simulink model "QD2_DroneStack_MPC"  (R2022b)
settings: Solver=ode1  StartTime=0.0  StopTime=inf  FixedStep=1/1000  RelTol=1e-3  EnableMultiTasking=on
InitFcn:
  | % QD2_DroneStack_MPC: rutas de la librería qd2_* y del mapeo de motores
  | qd2_d = fileparts(get_param(bdroot, 'FileName'));
  | for qd2_k = 1:4
  |     if exist(fullfile(qd2_d, 'lib', 'qd2_params.m'), 'file'), break; end
  |     qd2_d = fileparts(qd2_d);
  | end
  | addpath(fullfile(qd2_d, 'lib'));
  | addpath(fullfile(qd2_d, 'equipo2_original'));
  | clear qd2_d qd2_k
  | Motor_Mapping_7_Inch
model workspace (MAT data in the model file):
  target_system = 1
undefined symbols (not defined in the file): _Commander, _QDrone2, _Stabilizer, datetime, HIL, KT, lf, log_, m, Motor_Matrix, n, qc_get_step_size, s, saved_data
libraries: quarc_library x94, simulink x27, simulink_extras x9
(part 2 of 5)

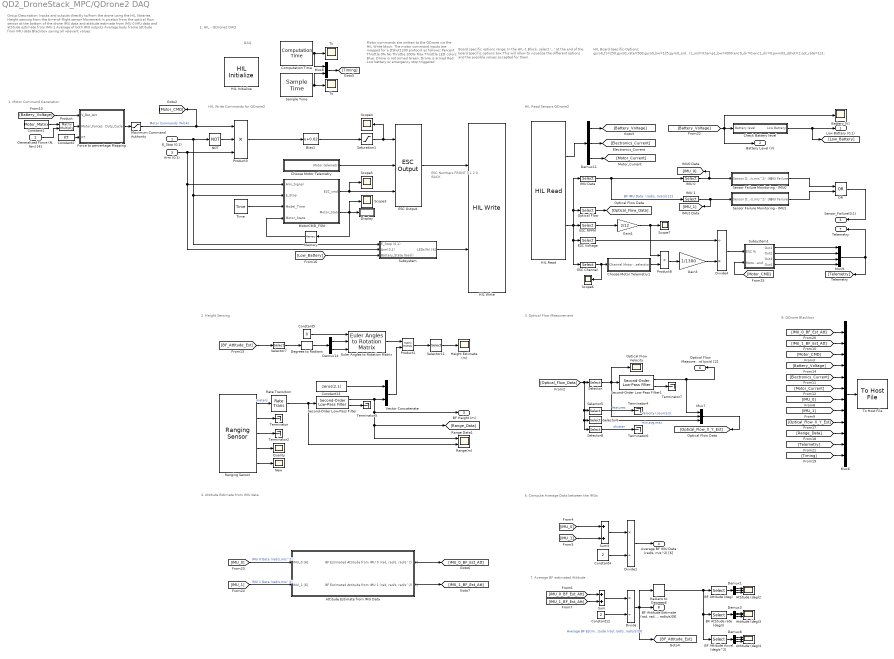
== system QD2_DroneStack_MPC/QDrone2 DAQ ==
  note: 4. Attitude Estimate from IMU data
  note: 1. Motor Command Generation
  note: HIL Write Commands for QDrone2
  note: HIL Read Sensors QDrone2
  note: ESC Numbers
      |
      | FRONT
      | 3 1
      |
      | 2 0
      | BACK
  note: 1. HIL - QDrone2 DAQ
  note: Group Description:
      |
      | Inputs and outputs directly to/from the drone using the HIL libraries.
      | Height sensing from the time-of-flight sensor
      | Movement in pixels/s from the optical flow sensor at the bottom of the drone
      | IMU data and attitude estimate from IMU 0
      | IMU data and attitude estimate from IMU 1
      | Average of both IMU outputs
      | Average body frame attitude from IMU data
      | Blackbox saving all relevant values
  note: DAQ
  note: HIL Board Specific-Options:
      | gyro0_fs=250;gyro0_rate=500;gyro0_bw=125;gyro0_ord=3;accel0_fs=16;accel0_rate=1000;accel0_bw=400;accel0_ord=3;temp0_bw=4000;gyro1_fs=250;gyro1_rate=500;gyro1_bw=125;gyro1_ord=3;accel1_fs=16;accel1_rate=1000;accel1_bw=400;accel1_ord=3;temp1_bw=4000;enc0_dir=0;enc1_dir=0;pwm03_dshot=1;opt_rate=121;
  note: Motor commands are written to the QDrone via the HIL Write block. The motor command inputs are mapped for a DShot1200 protocol as follows:
      |
      | Percent Throttle
      | 0% No Throttle
      | 100% Max Throttle
      |
      | LED colors:
      | Blue: Drone is not armed
      | Green: Drone is armed
      | Red: Low battery or emergency stop triggered
  note: Board specific options range:
      |
      | In the HIL-1 Block,
      | select '...' at the end of the board specific options box
      | This will allow to visualize the different options
      | and the possible values accepted for them.
  note: 2. Height Sensing
  note: 8. QDrone Blackbox
  note: 6. Compute Average Data between the IMUs
  note: 7. Average BF estimated Attitude
  note: 3. Optical Flow Measurement
  E_Stop (0,1) : Inport
  "Generalized Force (N, Nm) [4]" : Inport  Port=2
  Arm (0,1) : Inport  Port=3
  Attitude (deg)2 : Scope  NumInputPorts=3
  Attitude (deg)3 : Scope  NumInputPorts=3
  Attitude (deg)4 : Scope  NumInputPorts=3
  Attitude Estimate from IMU Data : Subsystem
  BF Attitude (deg) : Selector  InputPortWidth=9  IndexOptions=Index vector (dialog)  Indices=[1:3]  OutputSizes=1
  BF Attitude Accel (deg/s^2) : Selector  InputPortWidth=9  IndexOptions=Index vector (dialog)  Indices=[7:9]  OutputSizes=1
  BF Attitude rate (deg/s) : Selector  InputPortWidth=9  IndexOptions=Index vector (dialog)  Indices=[4:6]  OutputSizes=1
  Battery (V) : Scope
  Bias1 : Bias  Bias=0.02  SaturateOnIntegerOverflow=off
  Check Battery level : Subsystem
  Choose Motor Telemetry : Subsystem
  Choose Motor Telemetry1 : Subsystem
  Computation Time : quarc_library/Sources/Time/Computation Time  sample_time=qc_get_step_size  use_model=on  use_cpu_time=off
  Constant1 : Constant  Value=Motor_Matrix  OutDataTypeStr=double
  Constant12 : Constant  Value=2
  Constant13 : Constant  Value=zeros(2,1)
  Constant2 : Constant  Value=KT  OutDataTypeStr=double
  Constant4 : Constant  Value=2
  Constant5 : Constant  Value=0
  Degrees to Radians : simulink_extras/Transformations/Degrees to Radians
  Demux{1,3,8,11} (4 alike) : Demux  Outputs=3
  Demux14 : Demux  Outputs=2
  Display : Display
  Divide : Product  Inputs=*/
  Divide1 : Product  Inputs=*/
  Divide4 : Product  Inputs=/*
  ESC Channel : Selector  InputPortWidth=22  IndexOptions=Index vector (dialog)  Indices=[22]  OutputSizes=1
  ESC Output : quarc_library/Data Acquisition/Generic/Transformations/ESC Output  protocol=DShot (raw)  sign=Unsigned
      settings: AttributesFormatString=%<protocol>  SourceProductName=QUARC Targets
  ESC RPPM : Selector  InputPortWidth=22  IndexOptions=Index vector (dialog)  Indices=[20]  OutputSizes=1
  ESC Voltage : Selector  InputPortWidth=22  IndexOptions=Index vector (dialog)  Indices=[21]  OutputSizes=1
  Euler Angles to Rotation Matrix : quarc_library/Math Operations/Matrices/Euler Angles to Rotation Matrix  menu_order=Relative Z-X-Y
      settings: SourceProductName=QUARC Targets
  Force to percentage Mapping : MATLAB Function  TreatAsAtomicUnit=on
  Gain1 : Gain  Gain=2/12
  Gain3 : Gain  Gain=1/1300
  HIL Initialize : quarc_library/Data Acquisition/Generic/Configuration/HIL Initialize  object_name=HIL-1  board_type=qdrone2  board_number=0  board_options=gyro0_fs=250;gyro0_rate=500;gyro0_bw=125;gyro0_ord=3;accel0_fs=16;accel0_rate=1000;accel0_bw=400;accel0_ord=3;temp0_bw=4000;gyro1_fs=250;gyro1_rate=500;gyro1_bw=125;gyro1_ord=3;accel1_fs=16;accel1_rate=1000;accel1_bw=400;accel1_ord=3;temp1_bw=4000;enc0_dir=0;enc1_dir=0;pwm03_dshot=1;opt_rate=121;  exclusive=off  active=on  hardware_clocks=[]  clock_modes=[]  initial_clock_frequencies=[]  set_clock_params_at_start=off  set_clock_params_at_switch_in=off  set_clock_frequencies_at_start=off  set_clock_frequencies_at_switch_in=off  analog_input_channels=[0:4]  analog_input_configurations=[]  analog_input_maximums=[3.3]  analog_input_minimums=[0]  set_analog_input_params_at_start=off  set_analog_input_params_at_switch_in=off  analog_output_channels=[]  analog_output_maximums=[]  analog_output_minimums=[]  initial_analog_outputs=[]  final_analog_outputs=[]  watchdog_analog_outputs=[]  set_analog_output_params_at_start=off  set_analog_output_params_at_switch_in=off  set_analog_outputs_at_start=off  set_analog_outputs_at_switch_in=off  set_analog_outputs_at_terminate=off  set_analog_outputs_at_switch_out=off  set_analog_outputs_on_watchdog=off  digital_input_channels=[0:5]  digital_output_channels=[6:11]  digital_output_configuration=[]  initial_digital_outputs=[0]  final_digital_outputs=[0]  watchdog_digital_outputs=[0 0 0 0 0 0]  set_digital_output_params_at_start=off  set_digital_output_params_at_switch_in=off  set_digital_outputs_at_start=on  set_digital_outputs_at_switch_in=off  set_digital_outputs_at_terminate=on  set_digital_outputs_at_switch_out=off  set_digital_outputs_on_watchdog=off  encoder_channels=[0:1]  quadrature=[4]  encoder_filter_frequency=100e6/1  initial_encoder_counts=[0]  set_encoder_params_at_start=on  set_encoder_params_at_switch_in=off  set_encoder_counts_at_start=on  set_encoder_counts_at_switch_in=off  pwm_channels=[0:5]  pwm_modes=[6 6 6 6 0 0]  pwm_frequency=1.2e6  pwm_configuration=[0]  pwm_alignment=[0]  pwm_polarity=[1]  pwm_leading_deadband=[]  pwm_trailing_deadband=[]  initial_pwm_outputs=[0]  final_pwm_outputs=[0]  watchdog_pwm_outputs=[0]  set_pwm_params_at_start=on  set_pwm_params_at_switch_in=off  set_pwm_outputs_at_start=on  set_pwm_outputs_at_switch_in=off  set_pwm_outputs_at_terminate=on  set_pwm_outputs_at_switch_out=off  set_pwm_outputs_on_watchdog=off  other_output_channels=[]  initial_other_outputs=[0]  final_other_outputs=[0]  watchdog_other_outputs=[]  set_other_outputs_at_start=on  set_other_outputs_at_switch_in=off  set_other_outputs_at_terminate=on  set_other_outputs_at_switch_out=off  set_other_outputs_on_watchdog=off
  HIL Read : quarc_library/Data Acquisition/Generic/Immediate I//O/HIL Read  object_name=HIL-1  analog_channels=[3 1:2]  encoder_channels=[]  digital_channels=[]  other_channels=[3000:3002 4000:4002 3003:3005 4003:4005 17000:17006 17008:17009 17007]  sample_time=qc_get_step_size  active=on  vector_output=on  port_labels=channel numbers  data_type_mode=Inherit via back propagation  encoder_data_type=double  digital_data_type=boolean
  HIL Write : quarc_library/Data Acquisition/Generic/Immediate I//O/HIL Write  object_name=HIL-1  analog_channels=[]  pwm_channels=[0:3]  digital_channels=[6:11]  other_channels=[]  sample_time=-1  active=off  vector_input=on  port_labels=channel numbers
  Height Estimate (m) : Scope
  IMU 0 : Selector  InputPortWidth=12  IndexOptions=Index vector (dialog)  Indices=[1:6]  OutputSizes=1
  IMU 1 : Selector  InputPortWidth=12  IndexOptions=Index vector (dialog)  Indices=[7:12]  OutputSizes=1
  IMU Data : Selector  InputPortWidth=22  IndexOptions=Index vector (dialog)  Indices=[1:12]  OutputSizes=1
  "Maximum Command Authority " : Saturate  UpperLimit=[1 1 1 1]  LowerLimit=[0 0 0 0]
  Memory : Memory
  MotorCMD_FSM : MATLAB Function  TreatAsAtomicUnit=on
  Mux6 : Mux  Inputs=12
  Mux7 : Mux  Inputs=3
  Mux8 : Mux  Inputs=2
  Mux9 : Mux
  NOT : Logic  Operator=NOT  IconShape=distinctive  AllPortsSameDT=off  OutDataTypeStr=boolean
  New : Scope
  OR : Logic  Operator=OR  AllPortsSameDT=off  OutDataTypeStr=boolean
  Optical Flow : Selector  InputPortWidth=22  IndexOptions=Index vector (dialog)  Indices=[13:19]  OutputSizes=1
  Optical Flow Velocity : Scope
  Product : Product  Multiplication=Matrix(*)
  Product1 : Product  Multiplication=Matrix(*)
  Product3 : Product  Inputs=3
  Product8 : Product
  Quality : Scope
  Radians to Degrees6 : simulink_extras/Transformations/Radians to Degrees
  Range(m) : Scope  NumInputPorts=2
  Ranging Sensor : quarc_library/Devices/Third-Party/Sensors/Ranging Sensor  sensor_type=VL53L1X Time-of-flight  uri=i2c-cpu://localhost:0?address='0x29',baud='400000',memsize='512'  ranging_distance=Long  timing_budget=0.033  measurement_period=0.040  output_mode=Fixed-size output  samples_per_revolution=1300  max_distance=0.050  max_angle=5  sample_time=qc_get_step_size * ceil(1/121/ qc_get_step_size)  show_versions=off  active=on
      settings: SourceProductName=QUARC Targets
  Rate Transition : RateTransition
  Sample Time : quarc_library/Sources/Time/Sample Time  Priority=-99  sample_time=qc_get_step_size
  Saturation1 : Saturate  UpperLimit=1  LowerLimit=0
  Scope{3..7} (5 alike) : Scope
  Second-Order Low-Pass Filter : quarc_library/Continuous/Second-Order Low-Pass Filter  params_source=Internal (dialog parameters)  input_width=100  input_zeta=0.7  input_init=0
  Second-Order Low-Pass Filter1 : quarc_library/Continuous/Second-Order Low-Pass Filter  params_source=Internal (dialog parameters)  input_width=45  input_zeta=1.5  input_init=0
  Selector : Selector  InputPortWidth=7  IndexOptions=Index vector (dialog)  Indices=[1 2]  OutputSizes=1
  Selector11 : Selector  InputPortWidth=3  IndexOptions=Index vector (dialog)  Indices=[3]  OutputSizes=1
  Selector5 : Selector  InputPortWidth=7  IndexOptions=Index vector (dialog)  Indices=[3]  OutputSizes=1
  Selector6 : Selector  InputPortWidth=7  IndexOptions=Index vector (dialog)  Indices=[4 5 6]  OutputSizes=1
  Selector7 : Selector  InputPortWidth=9  IndexOptions=Index vector (dialog)  Indices=[1,2]  OutputSizes=1
  Selector8 : Selector  InputPortWidth=7  IndexOptions=Index vector (dialog)  Indices=[7]  OutputSizes=1
  Sensor Failure Monitoring - IMU0 : Subsystem
  Sensor Failure Monitoring - IMU1 : Subsystem
  Subsystem : Subsystem
  Subsystem1 : Subsystem
  Sum : Sum
  Sum3 : Sum
  Tc : Scope
  Terminator{,2,4..7} (6 alike) : Terminator
  Time : quarc_library/Sources/Time/Time  time_source=Wall clock  sample_time=qc_get_step_size
  To Host File : quarc_library/Sinks/To Host/To Host File  source=Specify via dialog (do not evaluate)  file_name=saved_data/%m/log_%{regexprep(char(datetime),' ','_')}_QDrone2.mat  variable_name=QDrone_data  decimation=1  sample_time=-1  file_format=MAT-file v.4  options=No header or footer  append=off  final_file_name=saved_data/QD2_DroneStack_MPC/log_22-Nov-2026_07-15-10_QDrone2.mat  encoding=Default  bitrate=2000000
  Ts : Scope
  Vector Concatenate : Concatenate
  Low Battery (0,1) : Outport
  Battery Level (V) : Outport  Port=2
  Sensor_Failure(0,1) : Outport  Port=3
  "Average BF IMU Data (rad/s, m/s^2) [6]" : Outport  Port=4
  "BF Height (m) " : Outport  Port=5
  Optical Flow Measurement (px/s) [2] : Outport  Port=6
  Telemetry : Outport  Port=7
  "BF Attitude Estimate (rad, rad/s, rad/s/s)[9]" : Outport  Port=8
  wires:
  Constant2/1 -> Force to percentage Mapping/3(KT)
  Constant1/1 -> Product/1
  "Generalized Force (N, Nm) [4]"/1 -> Product/2
  Product/1 -> Force to percentage Mapping/2(Motor_Forces)
  Force to percentage Mapping/1(Duty_Cycle) -> "Maximum Command Authority "/1
  "Maximum Command Authority "/1 -> Product3/1, [Motor_CMD]  "Motor Commands (%)[4]"
  [Battery_Voltage] -> Force to percentage Mapping/1(V_Bat_Act)
  Bias1/1 -> Saturation1/1
  ESC Voltage/1 -> Divide4/1
  IMU 0/1 -> Sensor Failure Monitoring - IMU0/1(Sensor Data (rad/s,m/s^2)  [6]), [IMU_0]
  OR/1 -> Sensor_Failure(0,1)/1
  Check Battery level/1(Low Battery) -> [Low_Battery], Low Battery (0,1)/1
  Optical Flow/1 -> [Optical_Flow_Data]
  IMU Data/1 -> IMU 0/1, IMU 1/1  "BF IMU Data  (rad/s, m/s/s)[12]"
  HIL Read/1 -> Demux11/1
  Gain1/1 -> Product8/1, Scope7/1
  NOT/1 -> Product3/2
  Memory/1 -> MotorCMD_FSM/4("Motor_State ")
  E_Stop (0,1)/1 -> Subsystem/1(E_Stop (0,1)), MotorCMD_FSM/2(E_Stop), NOT/1
  Subsystem/1(LEDs(%) [6]) -> HIL Write/2
  Demux11/2 -> [Electronics_Current]
  Sensor Failure Monitoring - IMU0/1(IMU Failure) -> OR/1
  ESC Output/1 -> HIL Write/1
  HIL Read/2 -> IMU Data/1, Optical Flow/1, ESC Voltage/1, ESC Channel/1, ESC RPPM/1
  [Battery_Voltage] -> Check Battery level/1(Battery level), Battery Level (V)/1, Battery (V)/1
  Demux11/3 -> [Motor_Current]
  IMU 1/1 -> [IMU_1], Sensor Failure Monitoring - IMU1/1(Sensor Data (rad/s,m/s^2)  [6])
  Choose Motor Telemetry1/1(Motor selection) -> Product8/2
  MotorCMD_FSM/2(Motor_State) -> Scope3/1, Display/1, Memory/1
  Gain3/1 -> Divide4/2
  Time/1 -> MotorCMD_FSM/3(Model_Time)
  Choose Motor Telemetry/1(Motor telemetry) -> ESC Output/2
  ESC Channel/1 -> Scope6/1, Choose Motor Telemetry1/1(Channel)
  Arm (0,1)/1 -> MotorCMD_FSM/1(Arm_Signal), Subsystem/2("Arm(0,1) "), Product3/3
  MotorCMD_FSM/1(ESC_cmd) -> Scope5/1, ESC Output/3
  Sensor Failure Monitoring - IMU1/1(IMU Failure) -> OR/2
  [Low_Battery] -> Subsystem/3(Battery_State (bool))
  ESC RPPM/1 -> Gain1/1
  Product8/1 -> Gain3/1
  Product3/1 -> Bias1/1
  Saturation1/1 -> ESC Output/1, Scope4/1
  Mux8/1 -> [Timing]
  Computation Time/1 -> Mux8/1, Tc/1
  Sample Time/1 -> Mux8/2, Ts/1
  Ranging Sensor/5 -> New/1
  [Range_Data] -> Mux6/10
  Selector5/1 -> Terminator4/1  "features"
  Mux7/1 -> [Optical_Flow_X_Y_Est]
  [Motor_CMD] -> Mux6/3
  Constant12/1 -> Divide/2
  Demux14/1 -> Euler Angles to Rotation Matrix/2
  Demux3/3 -> Attitude (deg)3/3
  Demux14/2 -> Euler Angles to Rotation Matrix/3
  [IMU_0_BF_Est_Att] -> Mux6/1
  [IMU_1_BF_Est_Att] -> Sum/2
  Mux9/1 -> [Telemetry], Telemetry/1
  [Optical_Flow_Data] -> Selector8/1, Selector6/1, Selector5/1, Selector/1
  BF Attitude Accel (deg/s^2)/1 -> Demux8/1
  Divide1/1 -> "Average BF IMU Data (rad/s, m/s^2) [6]"/1
  Subsystem1/4(Out4) -> Mux9/4
  [Timing] -> Mux6/12
  Selector6/1 -> Mux7/3  "min,avg,max"
  [Motor_CMD] -> Subsystem1/2(Motor command)
  [Telemetry] -> Mux6/11
  [IMU_1_BF_Est_Att] -> Mux6/2
  Constant13/1 -> Vector Concatenate/1
  [IMU_0] -> Sum3/1
  BF Attitude rate (deg/s)/1 -> Demux3/1
  Product1/1 -> Selector11/1
  [Motor_Current] -> Mux6/6
  Selector11/1 -> Height Estimate (m)/1
  Second-Order Low-Pass Filter/1 -> Vector Concatenate/2, [Range_Data], Range(m)/1, "BF Height (m) "/1
  Demux1/2 -> Attitude (deg)2/2
  Selector7/1 -> Degrees to Radians/1
  Constant5/1 -> Euler Angles to Rotation Matrix/1
  Second-Order Low-Pass Filter1/1 -> Mux7/1, Optical Flow Measurement (px/s) [2]/1
  Rate Transition/1 -> Range(m)/2, Second-Order Low-Pass Filter/1
  Subsystem1/3(Out3) -> Mux9/3
  Demux8/3 -> Attitude (deg)4/3
  Ranging Sensor/1 -> Rate Transition/1  "meters"
  Divide/1 -> "BF Attitude Estimate (rad, rad/s, rad/s/s)[9]"/1, [BF_Attitude_Est], Radians to Degrees6/1  "Average BF Estimated Attitude (rad, rad/s, rad/s/s)[9]"
  Degrees to Radians/1 -> Demux14/1
  Constant4/1 -> Divide1/2
  Euler Angles to Rotation Matrix/1 -> Product1/1
  [IMU_1] -> Sum3/2
  Demux1/3 -> Attitude (deg)2/3
  Demux8/2 -> Attitude (deg)4/2
  [IMU_1] -> Mux6/8
  [Optical_Flow_X_Y_Est] -> Mux6/9
  [BF_Attitude_Est] -> Selector7/1
  Ranging Sensor/4 -> Quality/1
  Subsystem1/1(Out1) -> Mux9/1
  Sum/1 -> Divide/1
  Vector Concatenate/1 -> Product1/2
  Demux3/1 -> Attitude (deg)3/1
  Selector8/1 -> Terminator6/1  "shutter"
  Radians to Degrees6/1 -> BF Attitude Accel (deg/s^2)/1, BF Attitude rate (deg/s)/1, BF Attitude (deg)/1
  Demux8/1 -> Attitude (deg)4/1
  Demux3/2 -> Attitude (deg)3/2
  Ranging Sensor/2 -> Terminator/1
  Ranging Sensor/3 -> Terminator2/1
  [IMU_0] -> Mux6/7
  Demux1/1 -> Attitude (deg)2/1
  [Battery_Voltage] -> Mux6/4
  Mux6/1 -> To Host File/1
  [Electronics_Current] -> Mux6/5
  [IMU_0_BF_Est_Att] -> Sum/1
  Divide4/1 -> Subsystem1/1(ESC %)
  BF Attitude (deg)/1 -> Demux1/1
  Sum3/1 -> Divide1/1
  Subsystem1/2(Out2) -> Mux9/2
  Selector/1 -> Second-Order Low-Pass Filter1/1, Mux7/2, Optical Flow Velocity/1  "Velocity (counts/s)"
  Demux11/1 -> [Battery_Voltage]
  Second-Order Low-Pass Filter/2 -> Terminator5/1
  Second-Order Low-Pass Filter1/2 -> Terminator7/1
  [IMU_0] -> Attitude Estimate from IMU Data/1(IMU_0 [6])  "IMU 0 Data (rad/s,m/s^2)"
  [IMU_1] -> Attitude Estimate from IMU Data/2(IMU_1 [6])  "IMU 1 Data (rad/s,m/s^2)"
  Attitude Estimate from IMU Data/1("BF Estimated Attitude from IMU 0 (rad, rad/s, rad/s^2) [9]") -> [IMU_0_BF_Est_Att]
  Attitude Estimate from IMU Data/2("BF Estimated Attitude from IMU 1 (rad, rad/s, rad/s^2) [9]") -> [IMU_1_BF_Est_Att]

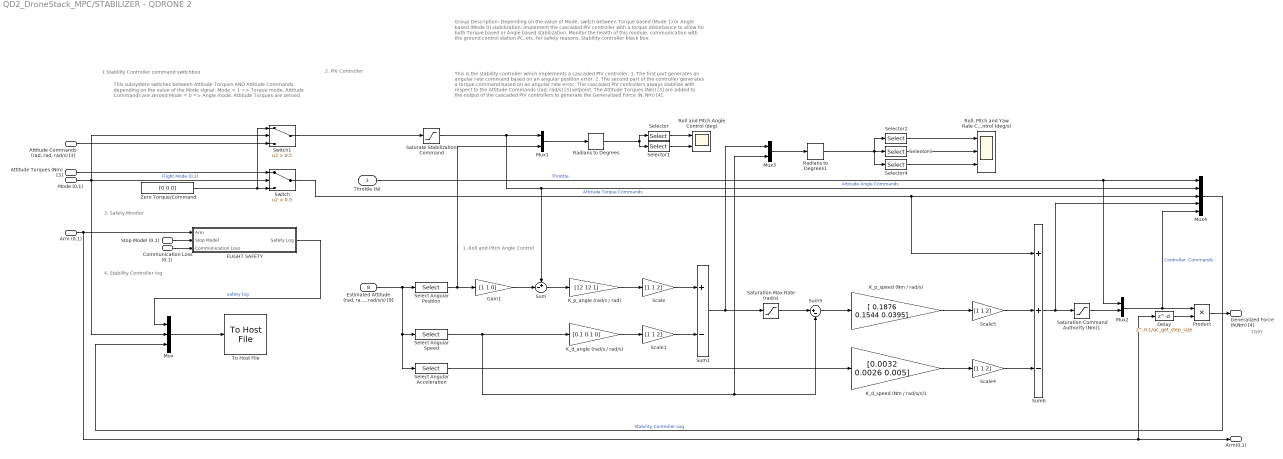
== system QD2_DroneStack_MPC/STABILIZER - QDRONE 2 ==
  note: 3. Safety Monitor
  note: This subsystem switches between Attitude Torques AND Attitude Commands depending on
      | the value of the Mode signal:
      | Mode = 1	=> 		Torque mode, Attitude Commands are zeroed
      | Mode = 0	=> 		Angle mode, Attitude Torques are zeroed
  note: This is the stability controller which implements a cascaded PIV controller.
      | 1. The first part generates an angular rate command based on an angular position error.
      | 2. The second part of the controller generates a torque command based on an angular rate error.
      |
      | The cascaded PIV controllers always stabilize with respect to the Attitude Commands (rad, rad/s) [3] setpoint. The Attitude Torques (Nm) [3] are added to the output of the cascaded PIV controllers to generate the Generalized Force (N, Nm) [4].
  note: 1. Roll and Pitch Angle Control
  note: TRPY
  note: Group Description:
      |
      | Depending on the value of Mode, switch between Torque based (Mode 1) or Angle based (Mode 0) stabilization.
      | Implement the cascaded PIV controller with a torque disturbance to allow for both Torque based or Angle based stabilization.
      | Monitor the health of this module, communication with the ground control station PC, etc. for safety reasons.
      | Stability controller black box.
  note: 1 Stability Controller command switchbox
  note: 4. Stability Controller log
  note: 2. PIV Controller
  Mode (0,1) : Inport
  Stop Model (0,1) : Inport  Port=2
  Throttle (N) : Inport  Port=3
  Attitude Torques (Nm) [3] : Inport  Port=4
  "Attitude Commands (rad, rad, rad/s) [3]" : Inport  Port=5
  Arm (0,1) : Inport  Port=6
  Communication Loss (0,1) : Inport  Port=7
  "Estimated Attitude (rad, rad/s, rad/s/s) [9]" : Inport  Port=8
  Delay : Delay  DelayLength=0.1/qc_get_step_size
  FLIGHT SAFETY : Subsystem
  Gain1 : Gain  Gain=[1 1 0]
  K_d_angle (rad/s / rad/s) : Gain  Gain=[0.1 0.1 0]
  K_d_speed (Nm / rad/s/s)1 : Gain  Gain="[0.0032    0.0026     0.005]"
  K_p_angle (rad/s / rad) : Gain  Gain=[12 12 1]
  K_p_speed (Nm / rad/s) : Gain  Gain="[ 0.1876    0.1544    0.0395]"
  Mux : Mux  Inputs=3
  Mux1 : Mux  Inputs=2
  Mux2 : Mux  Inputs=2
  Mux3 : Mux  Inputs=2
  Mux4 : Mux  Inputs=5
  Product : Product
  Radians to Degrees : simulink_extras/Transformations/Radians to Degrees
  Radians to Degrees1 : simulink_extras/Transformations/Radians to Degrees
  Roll and Pitch Angle Control (deg) : Scope  NumInputPorts=2
  "Roll, Pitch and Yaw Rate Control (deg/s)" : Scope  NumInputPorts=3
  Saturate Stabilization Command : Saturate  UpperLimit=[pi/4 pi/4 10*pi/18]  LowerLimit=[-pi/4 -pi/4 -10*pi/18]
  Saturation Command Authority (Nm)1 : Saturate  UpperLimit=[1.0915 0.8984 0.0984]  LowerLimit=-[1.0915 0.8984 0.0984]
  Saturation Max Rate (rad/s) : Saturate  UpperLimit=10*pi/3*[1 1 1]  LowerLimit=-10*pi/3*[1 1 1]
  Scale{,1,4..5} (4 alike) : Gain  Gain=[1 1 2]
  Select Angular Acceleration : Selector  InputPortWidth=9  IndexOptions=Index vector (dialog)  Indices=[7:9]  OutputSizes=1
  Select Angular Speed : Selector  InputPortWidth=9  IndexOptions=Index vector (dialog)  Indices=[4:6]  OutputSizes=1
  Select Angular Position : Selector  InputPortWidth=9  IndexOptions=Index vector (dialog)  Indices=[1:3]  OutputSizes=1
  Selector : Selector  InputPortWidth=6  IndexOptions=Index vector (dialog)  Indices=[1 4]  OutputSizes=1
  Selector1 : Selector  InputPortWidth=6  IndexOptions=Index vector (dialog)  Indices=[2 5]  OutputSizes=1
  Selector2 : Selector  InputPortWidth=6  IndexOptions=Index vector (dialog)  Indices=[1 4]  OutputSizes=1
  Selector3 : Selector  InputPortWidth=6  IndexOptions=Index vector (dialog)  Indices=[2 5]  OutputSizes=1
  Selector4 : Selector  InputPortWidth=6  IndexOptions=Index vector (dialog)  Indices=[3 6]  OutputSizes=1
  Sum : Sum  Inputs=+-|
  Sum1 : Sum  Inputs=+-
  Sum5 : Sum  Inputs=|+-
  Sum6 : Sum  Inputs=++-
  Switch : Switch  Criteria=u2 > Threshold  Threshold=0.5  SaturateOnIntegerOverflow=off  InputSameDT=off
  Switch1 : Switch  Criteria=u2 > Threshold  Threshold=0.5  SaturateOnIntegerOverflow=off  InputSameDT=off
  To Host File : quarc_library/Sinks/To Host/To Host File  source=Specify via dialog (do not evaluate)  file_name=saved_data/%m/log_%{regexprep(char(datetime),' ','_')}_Stabilizer.mat  variable_name=stabilizer_data  decimation=1  sample_time=-1  file_format=MAT-file v.5  options=No header or footer  append=off  final_file_name=saved_data/QD2_DroneStack_MPC/log_22-Nov-2026_07-15-10_Stabilizer.mat  encoding=Default  bitrate=2000000
  Zero Torque/Command : Constant  Value=[0 0 0]
  Generalized Force (N,Nm) [4] : Outport  VectorParamsAs1DForOutWhenUnconnected=off
  Arm(0,1) : Outport  Port=2  VectorParamsAs1DForOutWhenUnconnected=off
  wires:
  Scale1/1 -> Sum1/2
  Scale/1 -> Sum1/1
  Delay/1 -> Product/2
  Zero Torque/Command/1 -> Switch1/1, Switch/3
  Attitude Torques (Nm) [3]/1 -> Switch/1
  "Attitude Commands (rad, rad, rad/s) [3]"/1 -> Switch1/3
  Radians to Degrees/1 -> Selector1/1, Selector/1
  K_d_angle (rad/s / rad/s)/1 -> Scale1/1
  Selector2/1 -> "Roll, Pitch and Yaw Rate Control (deg/s)"/1
  Selector/1 -> Roll and Pitch Angle Control (deg)/1
  Select Angular Speed/1 -> Mux3/2, Sum5/2, K_d_angle (rad/s / rad/s)/1
  K_p_angle (rad/s / rad)/1 -> Scale/1
  Selector4/1 -> "Roll, Pitch and Yaw Rate Control (deg/s)"/3
  Switch1/1 -> Saturate Stabilization Command/1
  Gain1/1 -> Sum/2
  Selector3/1 -> "Roll, Pitch and Yaw Rate Control (deg/s)"/2
  Mux1/1 -> Radians to Degrees/1
  "Estimated Attitude (rad, rad/s, rad/s/s) [9]"/1 -> Select Angular Speed/1, Select Angular Acceleration/1, Select Angular Position/1
  Radians to Degrees1/1 -> Selector3/1, Selector4/1, Selector2/1
  Switch/1 -> Sum6/1, Mux4/3  "Attitude Torque Commands"
  Selector1/1 -> Roll and Pitch Angle Control (deg)/2
  Throttle (N)/1 -> Mux4/1, Mux2/1  "Throttle"
  Select Angular Position/1 -> Mux1/2, Gain1/1
  Mux2/1 -> Product/1, Mux4/5  "Controller  Commands"
  Saturate Stabilization Command/1 -> Mux4/2, Sum/1, Mux1/1  "Attitude Angle Commands"
  Sum1/1 -> Mux3/1, Saturation Max Rate (rad/s)/1
  Mux3/1 -> Radians to Degrees1/1
  Arm (0,1)/1 -> FLIGHT SAFETY/1(Arm), Delay/1, Arm(0,1)/1
  Sum/1 -> K_p_angle (rad/s / rad)/1
  FLIGHT SAFETY/1(Safety Log) -> Mux/1  "safety log"
  Mode (0,1)/1 -> Mux/2, Switch1/2, Switch/2  "Flight Mode (0,1)"
  Mux4/1 -> Mux/3  "Stability Controller Log"
  Mux/1 -> To Host File/1
  Communication Loss (0,1)/1 -> FLIGHT SAFETY/3(Communication Loss)
  Stop Model (0,1)/1 -> FLIGHT SAFETY/2(Stop Model)
  Product/1 -> Generalized Force (N,Nm) [4]/1
  Saturation Max Rate (rad/s)/1 -> Sum5/1
  Sum5/1 -> K_p_speed (Nm / rad/s)/1
  K_p_speed (Nm / rad/s)/1 -> Scale5/1
  K_d_speed (Nm / rad/s/s)1/1 -> Scale4/1
  Scale4/1 -> Sum6/3
  Select Angular Acceleration/1 -> K_d_speed (Nm / rad/s/s)1/1
  Sum6/1 -> Mux4/4, Saturation Command Authority (Nm)1/1
  Saturation Command Authority (Nm)1/1 -> Mux2/2
  Scale5/1 -> Sum6/2

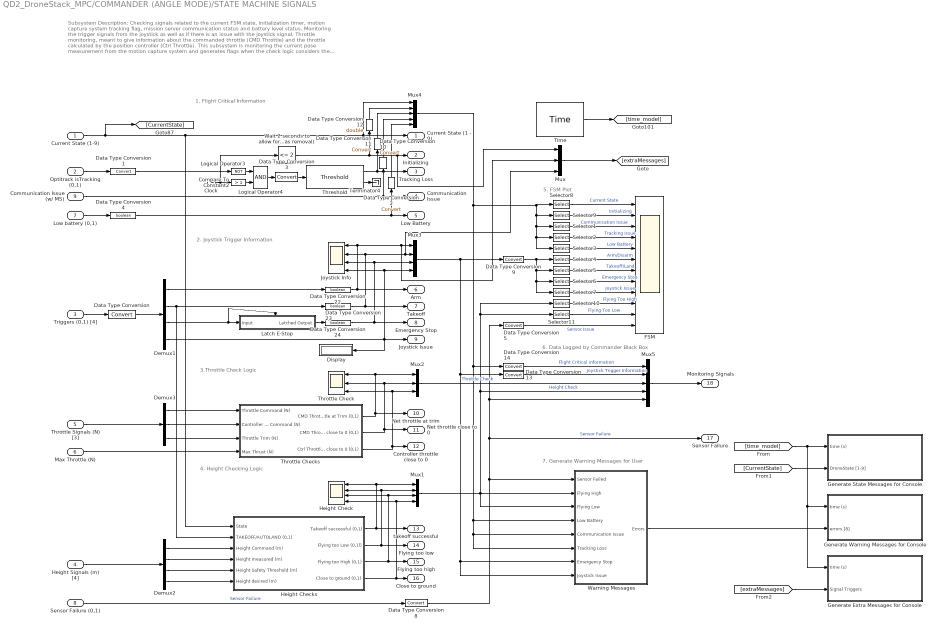
== system QD2_DroneStack_MPC/COMMANDER (ANGLE MODE)/STATE MACHINE SIGNALS ==
  note: Subsystem Description:
      | Checking signals related to the current FSM state, initialization timer, motion capture system tracking flag, mission server communication status and battery level status.
      | Monitoring the trigger signals from the joystick as well as if there is an issue with the joystick signal.
      | Throttle monitoring, meant to give information about the commanded throttle (CMD Throttle) and the throttle calculated by the position controller (Ctrl Throttle).
      | This subsystem is monitoring the current pose measurement from the motion capture system and generates flags when the check logic considers the QDrone flying to close to ground, too high or too low as well as generate a successful take off flag.
      | A subset of the FSM monitoring signals are shown using this scope. These signals are what Quanser considers importnat for flight.
      | FSM signals sent to the blackbox for post flight monitoring.
      | Error message generation based on flags generated by the FSM signal checks.
  note: 7. Generate Warning Messages for User
  note: 5. FSM Plot
  note: 6. Data Logged by Commander Black Box
  note: 1. Flight Critical Information
  note: 2. Joystick Trigger Information
  note: 3.Throttle Check Logic
  note: 4. Height Checking Logic
  Current State (1-9) : Inport
  "Optitrack isTracking (0,1)  " : Inport  Port=2
  Triggers (0,1) [4] : Inport  Port=3
  Height Signals (m) [4] : Inport  Port=4
  Throttle Signals (N) [3] : Inport  Port=5
  "Max Throttle (N) " : Inport  Port=6
  Low battery (0,1) : Inport  Port=7
  Sensor Failure (0,1) : Inport  Port=8
  Communication Issue (w/ MS) : Inport  Port=9
  Clock : Clock
  Compare To Constant2 : simulink/Logic and Bit Operations/Compare To Constant  relop=>  const=1  OutDataTypeStr=boolean
  Data Type Conversion{,1..3,5,8..11,13..14} (11 alike) : DataTypeConversion  SaturateOnIntegerOverflow=off  RndMeth=Floor
  Data Type Conversion12 : DataTypeConversion  OutDataTypeStr=double  SaturateOnIntegerOverflow=off  RndMeth=Floor
  Data Type Conversion{4,22..24} (4 alike) : DataTypeConversion  OutDataTypeStr=boolean  SaturateOnIntegerOverflow=off  RndMeth=Floor
  Demux1 : Demux  Outputs=[1 1 1 1]
  Demux2 : Demux
  Demux3 : Demux  Outputs=3
  Display : Display
  FSM : Scope  NumInputPorts=12
  Generate Extra Messages for Console : Subsystem
  Generate State Messages for Console : Subsystem
  Generate Warning Messages for Console : Subsystem
  "Height Check " : Scope  NumInputPorts=4
  Height Checks : Subsystem
  Joystick Info : Scope  NumInputPorts=4
  Latch E-Stop : Subsystem  TreatAsAtomicUnit=on
  Logical Operator3 : Logic  Operator=NOT  AllPortsSameDT=off  OutDataTypeStr=boolean
  Logical Operator4 : Logic  AllPortsSameDT=off  OutDataTypeStr=boolean
  Mux : Mux  Inputs=3
  Mux1 : Mux  Inputs=[1 1 1 1]
  Mux2 : Mux  Inputs=[1 1 1]
  Mux3 : Mux  Inputs=[1 1 1 1]
  Mux4 : Mux  Inputs=[1 1 1 1 1]
  Mux5 : Mux  Inputs=[5 4 3 4 1]
  Selector1 : Selector  InputPortWidth=5  IndexOptions=Index vector (dialog)  Indices=4  OutputSizes=1
  Selector10 : Selector  InputPortWidth=4  IndexOptions=Index vector (dialog)  Indices=3  OutputSizes=1
  Selector11 : Selector  InputPortWidth=4  IndexOptions=Index vector (dialog)  Indices=2  OutputSizes=1
  Selector2 : Selector  InputPortWidth=5  IndexOptions=Index vector (dialog)  Indices=3  OutputSizes=1
  Selector3 : Selector  InputPortWidth=5  IndexOptions=Index vector (dialog)  Indices=5  OutputSizes=1
  Selector4 : Selector  InputPortWidth=4  IndexOptions=Index vector (dialog)  Indices=1  OutputSizes=1
  Selector5 : Selector  InputPortWidth=4  IndexOptions=Index vector (dialog)  Indices=2  OutputSizes=1
  Selector6 : Selector  InputPortWidth=4  IndexOptions=Index vector (dialog)  Indices=3  OutputSizes=1
  Selector7 : Selector  InputPortWidth=4  IndexOptions=Index vector (dialog)  Indices=4  OutputSizes=1
  Selector8 : Selector  InputPortWidth=5  IndexOptions=Index vector (dialog)  Indices=1  OutputSizes=1
  Selector9 : Selector  InputPortWidth=5  IndexOptions=Index vector (dialog)  Indices=2  OutputSizes=1
  Terminator4 : Terminator
  Threshold : quarc_library/Discontinuities/Threshold  operator=>=  param_src=Specify via dialog  threshold=0.5  duration=0.2
      settings: SourceProductName=QUARC Targets
  Throttle Check : Scope  NumInputPorts=3
  Throttle Checks : Subsystem
  Time : quarc_library/Sources/Time/Time  time_source=Wall clock  sample_time=qc_get_step_size
  "Wait 2 seconds to allow for initialization (e.g., bias removal)" : simulink/Logic and Bit Operations/Compare To Constant  relop=<=  const=2  OutDataTypeStr=boolean
  Warning Messages : Subsystem
  "Current State (1 - 9)  " : Outport  VectorParamsAs1DForOutWhenUnconnected=off
  Initializing : Outport  Port=2  VectorParamsAs1DForOutWhenUnconnected=off
  Tracking Loss : Outport  Port=3  VectorParamsAs1DForOutWhenUnconnected=off
  Communication Issue : Outport  Port=4  VectorParamsAs1DForOutWhenUnconnected=off
  Low Battery : Outport  Port=5  VectorParamsAs1DForOutWhenUnconnected=off
  Arm : Outport  Port=6  VectorParamsAs1DForOutWhenUnconnected=off
  Takeoff : Outport  Port=7  VectorParamsAs1DForOutWhenUnconnected=off
  Emergency Stop : Outport  Port=8  VectorParamsAs1DForOutWhenUnconnected=off
  "Joystick Issue " : Outport  Port=9  VectorParamsAs1DForOutWhenUnconnected=off
  Net throttle at trim : Outport  Port=10  VectorParamsAs1DForOutWhenUnconnected=off
  Net throttle close to 0 : Outport  Port=11  VectorParamsAs1DForOutWhenUnconnected=off
  Controller throttle close to 0 : Outport  Port=12  VectorParamsAs1DForOutWhenUnconnected=off
  takeoff successful : Outport  Port=13  VectorParamsAs1DForOutWhenUnconnected=off
  Flying too low : Outport  Port=14  VectorParamsAs1DForOutWhenUnconnected=off
  Flying too high : Outport  Port=15  VectorParamsAs1DForOutWhenUnconnected=off
  Close to ground : Outport  Port=16  VectorParamsAs1DForOutWhenUnconnected=off
  "  Sensor Failure" : Outport  Port=17  VectorParamsAs1DForOutWhenUnconnected=off
  Monitoring Signals : Outport  Port=18  VectorParamsAs1DForOutWhenUnconnected=off
  wires:
  Triggers (0,1) [4]/1 -> Data Type Conversion/1
  Demux2/1 -> Height Checks/3(Height Command (m))
  Demux3/1 -> Throttle Checks/1(Throttle Command (N))
  Height Signals (m) [4]/1 -> Demux2/1
  Demux2/4 -> Height Checks/6(Height desired (m))
  Throttle Signals (N) [3]/1 -> Demux3/1
  Demux1/1 -> Data Type Conversion22/1
  Throttle Checks/2(CMD Throttle close to 0 (0,1)) -> Mux2/2, Throttle Check/2, Net throttle close to 0/1
  Height Checks/1(Takeoff successful (0,1)) -> takeoff successful/1, "Height Check "/1, Mux1/1
  Demux2/3 -> Height Checks/5(Height Safety Threshold (m))
  Demux1/2 -> Data Type Conversion23/1, Height Checks/2(TAKEOFF/AUTOLAND (0,1))
  Demux2/2 -> Height Checks/4(Height measured (m))
  Demux3/2 -> Throttle Checks/2(Controller Throttle Command (N))
  Demux3/3 -> Throttle Checks/3(Throttle Trim (N))
  Throttle Checks/1(CMD Throttle at Trim (0,1)) -> Net throttle at trim/1, Mux2/1, Throttle Check/1
  Height Checks/3(Flying too High (0,1)) -> Mux1/3, "Height Check "/3, Flying too high/1
  Height Checks/4(Close to ground (0,1)) -> "Height Check "/4, Mux1/4, Close to ground/1
  Data Type Conversion/1 -> Demux1/1
  Low battery (0,1)/1 -> Data Type Conversion4/1
  Height Checks/2(Flying too Low (0,1l)) -> Flying too low/1, Mux1/2, "Height Check "/2
  Sensor Failure (0,1)/1 -> Data Type Conversion8/1  "Sensor Failure"
  Data Type Conversion1/1 -> Logical Operator3/1
  Data Type Conversion3/1 -> Threshold/1
  Compare To Constant2/1 -> Logical Operator4/2
  Clock/1 -> "Wait 2 seconds to allow for initialization (e.g., bias removal)"/1, Compare To Constant2/1
  Logical Operator4/1 -> Data Type Conversion3/1
  Threshold/2 -> Terminator4/1
  Logical Operator3/1 -> Logical Operator4/1
  "Optitrack isTracking (0,1)  "/1 -> Data Type Conversion1/1
  Latch E-Stop/1(Latched Output) -> Data Type Conversion24/1
  Demux1/3 -> Latch E-Stop/1(Input), Latch E-Stop/Trigger
  Selector9/1 -> FSM/2  "Initializing"
  Selector1/1 -> FSM/3  "Communication Issue"
  Selector2/1 -> FSM/4  "Tracking Issue"
  Selector3/1 -> FSM/5  "Low Battery"
  Selector4/1 -> FSM/6  "Arm/Disarm"
  Selector5/1 -> FSM/7  "Takeoff/Land"
  Selector6/1 -> FSM/8  "Emergency Stop"
  Selector7/1 -> FSM/9  "Joystick Issue"
  Data Type Conversion5/1 -> FSM/12  "Sensor Issue"
  Selector10/1 -> FSM/10  "Flying Too High"
  Selector11/1 -> FSM/11  "Flying Too Low"
  Data Type Conversion24/1 -> Joystick Info/3, Mux3/3, Emergency Stop/1
  Data Type Conversion23/1 -> Joystick Info/2, Mux/3, Mux3/2, Takeoff/1
  Data Type Conversion22/1 -> Joystick Info/1, Mux/2, Mux3/1, Arm/1
  Data Type Conversion4/1 -> Low Battery/1, Data Type Conversion2/1
  Demux1/4 -> Display/1, Joystick Info/4, Mux3/4, "Joystick Issue "/1
  Communication Issue (w/ MS)/1 -> Communication Issue/1, Data Type Conversion10/1
  Threshold/1 -> Tracking Loss/1, Data Type Conversion11/1
  Mux5/1 -> Monitoring Signals/1
  Mux1/1 -> Warning Messages/3(Flying Low), Warning Messages/2(Flying High), Selector11/1, Selector10/1, Mux5/4  "Height Check"
  Mux2/1 -> Mux5/3  "Throttle Check"
  Mux3/1 -> Data Type Conversion9/1, Warning Messages/7("Emergency Stop "), Warning Messages/8(Joystick Issue), Data Type Conversion13/1
  Mux4/1 -> Warning Messages/4(Low Battery), Warning Messages/5(Communication Issue), Warning Messages/6(Tracking Loss), Data Type Conversion14/1, Selector3/1, Selector2/1, Selector1/1, Selector9/1, Selector8/1
  Throttle Checks/3(Ctrl Throttle close to 0 (0,1)) -> Mux2/3, Throttle Check/3, Controller throttle close to 0/1
  Data Type Conversion9/1 -> Selector4/1, Selector5/1, Selector7/1, Selector6/1
  Data Type Conversion8/1 -> "  Sensor Failure"/1, Data Type Conversion5/1, Mux5/5, Warning Messages/1(Sensor Failed)  "Sensor Failure"
  Current State (1-9)/1 -> [CurrentState], Mux4/1, "Current State (1 - 9)  "/1, Height Checks/1(State)
  Selector8/1 -> FSM/1  "Current State"
  Data Type Conversion2/1 -> Mux4/5
  Data Type Conversion10/1 -> Mux4/4
  Data Type Conversion11/1 -> Mux4/3
  Data Type Conversion12/1 -> Mux4/2
  Data Type Conversion13/1 -> Mux5/2  "Joystick Trigger Information"
  Data Type Conversion14/1 -> Mux5/1  "Flight Critical information"
  "Wait 2 seconds to allow for initialization (e.g., bias removal)"/1 -> Data Type Conversion12/1, Mux/1, Initializing/1
  "Max Throttle (N) "/1 -> Throttle Checks/4(Max Thrust (N))
  Time/1 -> [time_model]
  [time_model] -> Generate Warning Messages for Console/1(time (s)), Generate Extra Messages for Console/1(time (s)), Generate State Messages for Console/1(time (s))
  [CurrentState] -> Generate State Messages for Console/2(DroneState [1-9])
  Warning Messages/1(Errors) -> Generate Warning Messages for Console/2(errors [8])
  Mux/1 -> [extraMessages]
  [extraMessages] -> Generate Extra Messages for Console/2(Signal Triggers)

== system QD2_DroneStack_MPC/COMMANDER (ANGLE MODE)/Signal Smoothing ==
  "High Frequency Controller Commands (N,rad, rad/s)[4]" : Inport
  Constant4 : Constant
  Constant5 : Constant  Value=100
  Mux : Mux  Inputs=2
  Second-Order Low-Pass Filter : quarc_library/Continuous/Second-Order Low-Pass Filter  params_source=External (input ports)  input_width=60  input_zeta=1  input_init=0
  Selector1 : Selector  InputPortWidth=4  IndexOptions=Index vector (dialog)  Indices=[3:4]  OutputSizes=1
  Selector3 : Selector  InputPortWidth=4  IndexOptions=Index vector (dialog)  Indices=[1:2]  OutputSizes=1
  Terminator : Terminator
  "Smoothed Controller Commands (N,rad, rad/s)[4]" : Outport
  wires:
  "High Frequency Controller Commands (N,rad, rad/s)[4]"/1 -> Selector1/1, Selector3/1
  Mux/1 -> "Smoothed Controller Commands (N,rad, rad/s)[4]"/1
  Selector1/1 -> Mux/2
  Second-Order Low-Pass Filter/1 -> Mux/1
  Selector3/1 -> Second-Order Low-Pass Filter/4, Second-Order Low-Pass Filter/1
  Constant4/1 -> Second-Order Low-Pass Filter/3
  Constant5/1 -> Second-Order Low-Pass Filter/2
  Second-Order Low-Pass Filter/2 -> Terminator/1

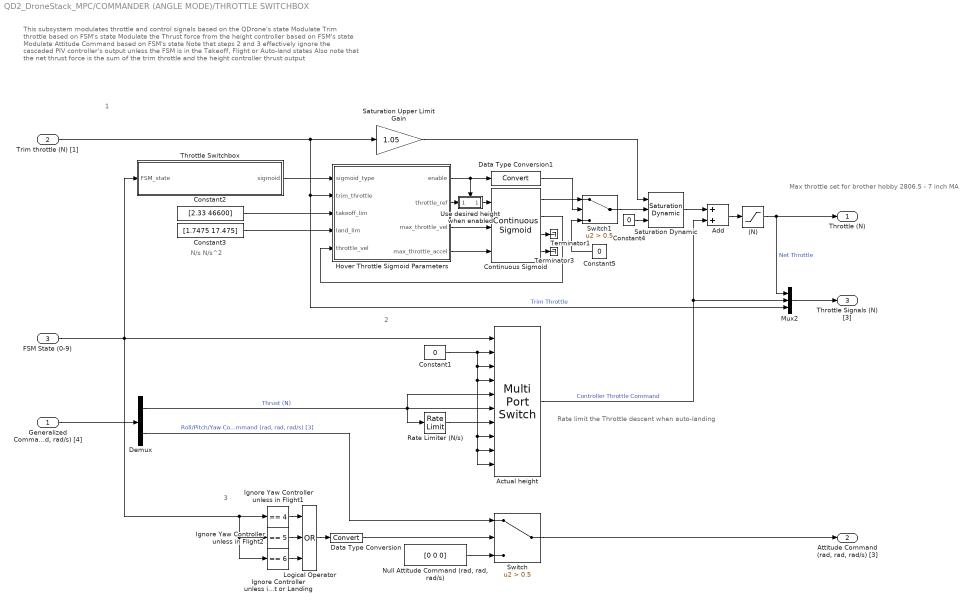
== system QD2_DroneStack_MPC/COMMANDER (ANGLE MODE)/THROTTLE SWITCHBOX  ==
  note: Max throttle set for brother hobby 2806.5 - 7 inch MA
  note: 3
  note: 2
  note: 1
  note: Rate limit the Throttle descent when auto-landing
  note: This subsystem modulates throttle and control signals based on the QDrone's state
      | Modulate Trim throttle based on FSM's state
      | Modulate the Thrust force from the height controller based on FSM's state
      | Modulate Attitude Command based on FSM's state
      |
      | Note that steps 2 and 3 effectively ignore the cascaded PIV controller's output unless the FSM is in the Takeoff, Flight or Auto-land states
      | Also note that the net thrust force is the sum of the trim throttle and the height controller thrust output
  note: N/s N/s^2
  "Generalized Command (N, rad, rad, rad/s) [4]" : Inport
  Trim throttle (N) [1] : Inport  Port=2
  FSM State (0-9) : Inport  Port=3
  (N) : Saturate  UpperLimit=58  LowerLimit=0
  Actual height : MultiPortSwitch  Inputs=9  SaturateOnIntegerOverflow=off  InputSameDT=off
  Add : Sum
  Constant1 : Constant  Value=0
  Constant2 : Constant  Value=[2.33 46600]
  Constant3 : Constant  Value=[1.7475 17.475]
  Constant4 : Constant  Value=0
  Constant5 : Constant  Value=0
  Continuous Sigmoid : quarc_library/Sources/Sigmoids/Continuous Sigmoid  params_source=External (input ports)  max_velocity=2  max_acceleration=10  initial_position=0  initial_velocity=0  hold_off=0.5  input_sample_time=-1  output_sample_time=qc_get_step_size
      settings: SourceProductName=QUARC Targets
  Data Type Conversion : DataTypeConversion  SaturateOnIntegerOverflow=off  RndMeth=Floor
  Data Type Conversion1 : DataTypeConversion  SaturateOnIntegerOverflow=off  RndMeth=Floor
  Demux : Demux  Outputs=[1 3]
  Hover Throttle Sigmoid Parameters : MATLAB Function  TreatAsAtomicUnit=on
  "Ignore Controller unless in Takeoff, Flight or Landing" : simulink/Logic and Bit Operations/Compare To Constant  relop===  const=6  OutDataTypeStr=boolean
  Ignore Yaw Controller unless in Flight1 : simulink/Logic and Bit Operations/Compare To Constant  relop===  const=4  OutDataTypeStr=boolean
  Ignore Yaw Controller unless in Flight2 : simulink/Logic and Bit Operations/Compare To Constant  relop===  const=5  OutDataTypeStr=boolean
  Logical Operator : Logic  Operator=OR  Inputs=3  AllPortsSameDT=off  OutDataTypeStr=boolean
  Mux2 : Mux  Inputs=3
  "Null Attitude Command (rad, rad, rad/s)" : Constant  Value=[0 0 0]
  Rate Limiter (N/s) : RateLimiter  RisingSlewLimit=100  FallingSlewLimit=-100  SampleTimeMode=inherited
  Saturation Dynamic : simulink/Discontinuities/Saturation Dynamic  OutMin=[]  OutMax=[]  OutDataTypeStr=Inherit: Same as second input  OutDataType=fixdt(1, 16)  OutScaling=2^-10  DoSatur=off
  Saturation Upper Limit Gain : Gain  Gain=1.05
  Switch : Switch  Criteria=u2 > Threshold  Threshold=0.5  SaturateOnIntegerOverflow=off  InputSameDT=off
  Switch1 : Switch  Criteria=u2 > Threshold  Threshold=0.5  SaturateOnIntegerOverflow=off  InputSameDT=off
  Terminator1 : Terminator
  Terminator3 : Terminator
  Throttle Switchbox : MATLAB Function  TreatAsAtomicUnit=on
  Use desired height when enabled : Subsystem  TreatAsAtomicUnit=on
  Throttle (N) : Outport  VectorParamsAs1DForOutWhenUnconnected=off
  "Attitude Command (rad, rad, rad/s) [3]" : Outport  Port=2  VectorParamsAs1DForOutWhenUnconnected=off
  Throttle Signals (N) [3] : Outport  Port=3  VectorParamsAs1DForOutWhenUnconnected=off
  wires:
  Actual height/1 -> Mux2/2, Add/2  "Controller Throttle Command"
  Add/1 -> (N)/1
  (N)/1 -> Mux2/1, Throttle (N)/1  "Net Throttle"
  "Generalized Command (N, rad, rad, rad/s) [4]"/1 -> Demux/1
  Mux2/1 -> Throttle Signals (N) [3]/1
  Ignore Yaw Controller unless in Flight2/1 -> Logical Operator/2
  Data Type Conversion/1 -> Switch/2
  "Null Attitude Command (rad, rad, rad/s)"/1 -> Switch/3
  Ignore Yaw Controller unless in Flight1/1 -> Logical Operator/1
  Demux/2 -> Switch/1  "Roll/Pitch/Yaw Command (rad, rad, rad/s) [3]"
  FSM State (0-9)/1 -> Actual height/1, "Ignore Controller unless in Takeoff, Flight or Landing"/1, Ignore Yaw Controller unless in Flight2/1, Ignore Yaw Controller unless in Flight1/1, Throttle Switchbox/1(FSM_state)
  "Ignore Controller unless in Takeoff, Flight or Landing"/1 -> Logical Operator/3
  Logical Operator/1 -> Data Type Conversion/1
  Demux/1 -> Actual height/6, Rate Limiter (N/s)/1, Actual height/5  "Thrust (N)"
  Continuous Sigmoid/2 -> Hover Throttle Sigmoid Parameters/5(throttle_vel)
  Constant4/1 -> Saturation Dynamic/3
  Saturation Dynamic/1 -> Add/1
  Constant3/1 -> Hover Throttle Sigmoid Parameters/4(land_lim)
  Switch1/1 -> Saturation Dynamic/2
  Trim throttle (N) [1]/1 -> Mux2/3, Hover Throttle Sigmoid Parameters/2(trim_throttle), Saturation Upper Limit Gain/1  "Trim Throttle"
  Throttle Switchbox/1(sigmoid) -> Hover Throttle Sigmoid Parameters/1(sigmoid_type)
  Saturation Upper Limit Gain/1 -> Saturation Dynamic/1
  Constant2/1 -> Hover Throttle Sigmoid Parameters/3(takeoff_lim)
  Hover Throttle Sigmoid Parameters/4(max_throttle_accel) -> Continuous Sigmoid/3
  Continuous Sigmoid/1 -> Switch1/1
  Continuous Sigmoid/4 -> Terminator3/1
  Hover Throttle Sigmoid Parameters/3(max_throttle_vel) -> Continuous Sigmoid/2
  Data Type Conversion1/1 -> Switch1/2
  Hover Throttle Sigmoid Parameters/1(enable) -> Data Type Conversion1/1, Use desired height when enabled/Enable
  Continuous Sigmoid/3 -> Terminator1/1
  Use desired height when enabled/1(Out1) -> Continuous Sigmoid/1
  Hover Throttle Sigmoid Parameters/2(throttle_ref) -> Use desired height when enabled/1(h_d (m) [1])
  Constant5/1 -> Switch1/3
  Switch/1 -> "Attitude Command (rad, rad, rad/s) [3]"/1
  Constant1/1 -> Actual height/8, Actual height/10, Actual height/9, Actual height/4, Actual height/3, Actual height/2
  Rate Limiter (N/s)/1 -> Actual height/7

== system QD2_DroneStack_MPC/Communication/Detect Communication Loss ==
  note: Stream Loss: Check if the state is 2 and error is positive (error codes are negative). Otherwise issue a communication error.
      | OR
      | Data Loss: Check if the data is stale for a while (this is required because a connected stream may publish no new data). If stale, issue a communication error.
  State : Inport
  Error : Inport  Port=2
  Data Out : Inport  Port=3
  Clock1 : Clock
  Communication Loss : Scope  NumInputPorts=2
  Data Type Conversion4 : DataTypeConversion  SaturateOnIntegerOverflow=off  RndMeth=Floor
  Grab mission server time to detect flat lines : Selector  IndexOptions=Index vector (dialog)  Indices=[16]  OutputSizes=1
  Logical Operator4 : Logic  Operator=OR  AllPortsSameDT=off  OutDataTypeStr=boolean
  MATLAB Function : MATLAB Function  TreatAsAtomicUnit=on
  Terminator3 : Terminator
  Terminator5 : Terminator
  Threshold1 : quarc_library/Discontinuities/Threshold  operator=>=  param_src=Specify via dialog  threshold=0.5  duration=0.1
      settings: SourceProductName=QUARC Targets
  Threshold2 : quarc_library/Discontinuities/Threshold  operator=>=  param_src=Specify via dialog  threshold=0.5  duration=0.5
      settings: SourceProductName=QUARC Targets
  Communication Issue : Outport  VectorParamsAs1DForOutWhenUnconnected=off
  wires:
  Threshold2/1 -> Communication Loss/2, Logical Operator4/2
  Logical Operator4/1 -> Data Type Conversion4/1
  Threshold1/2 -> Terminator3/1
  MATLAB Function/2(data_loss) -> Threshold2/1
  MATLAB Function/1(stream_connection_loss) -> Threshold1/1
  Clock1/1 -> MATLAB Function/1(time)
  Threshold2/2 -> Terminator5/1
  Threshold1/1 -> Communication Loss/1, Logical Operator4/1
  Grab mission server time to detect flat lines/1 -> MATLAB Function/4(ms_time)
  Data Out/1 -> Grab mission server time to detect flat lines/1
  State/1 -> MATLAB Function/2(state)
  Error/1 -> MATLAB Function/3(error)
  Data Type Conversion4/1 -> Communication Issue/1
